simulink model "Model_XInput_wFeedback_Masked"  (R2023a)
settings: Solver=FixedStepAuto  StartTime=0.0  StopTime=100  FixedStep=0.01  RelTol=1e-3
settings Model: Creator=Mathias Voigt  LastModifiedBy=FIRSTMentor
settings SolverCC: AlgebraicLoopSolver=TrustRegion
settings DebuggingCC: UnconnectedInputMsg=warning  UnconnectedOutputMsg=warning  UnconnectedLineMsg=warning
settings ModelReferenceCC: EnableRefExpFcnMdlSchedulingChecks=on
settings SFSimCC: CustomCodeUndefinedFunction=UseInterfaceOnly

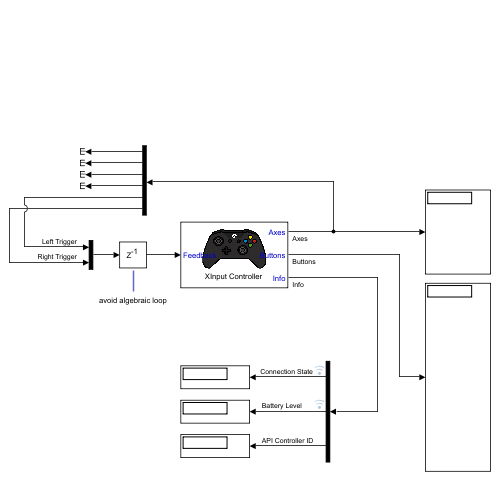
[thumbnail: Simulink's stored preview of the top-level diagram]
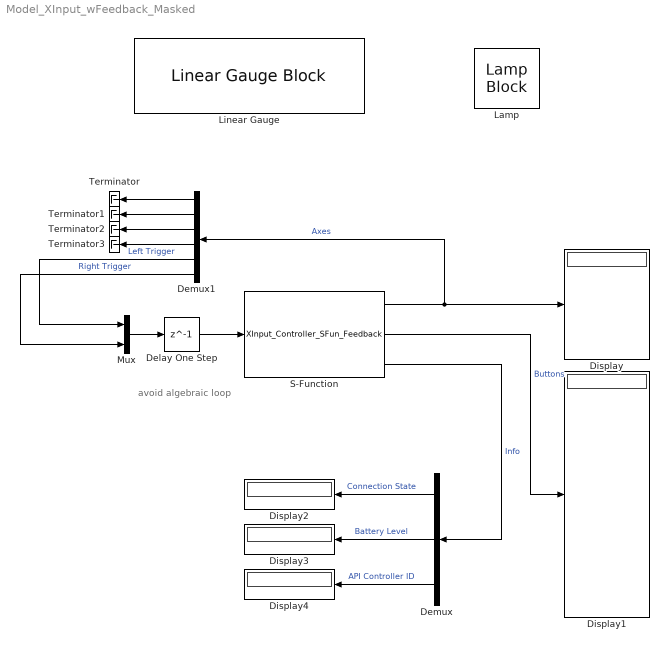
== system Model_XInput_wFeedback_Masked ==
  note: avoid algebraic loop
  Delay One Step : Delay  DelayLength=1
  Demux : Demux  Outputs=3
  Demux1 : Demux  Outputs=6
  Display{,1..4} (5 alike) : Display
  Lamp : LampBlock
  Linear Gauge : LinearGaugeBlock  TickInterval=25
  Mux : Mux  Inputs=2
  S-Function : S-Function  FunctionName=XInput_Controller_SFun_Feedback  Parameters=1  SFunctionDeploymentMode=off  EnableBusSupport=off  mask(XInput Controller (with Feedback)){ControllerID=1}
      mask help:
      | This Block will allow you to use XInput Controllers in Simulink.
      | XInput is the most Supported API.
      | Works with XBOX 360 and XBOX ONE Controllers.
      |
      | Use 'DEMUX' to access Signals
      | Output_1 [1x6]
      |   Analog Left X, Analog Left Y,
      |   Analog Right X, Analog Right Y,
      |   Left Trigger, Right Trigger
      | Output_2 [1x14]
      |   Up, Down, Left, Right,
      |   Start, Back, Left Stick, Right Stick,
      |   Left Shoulder, Right Shoulder,
      |   A, B, X, Y
      | Output_3 [1x3]
      |   Connection State, Battery Level (1-4), Controller ID
      | Input_1 [1x2]
      |   Left Motor, Right Motor (Force Feedback)
      mask init:
      | ControllerID;   
      | blk = gcb; 
      | get_String = get_param(blk,'ControllerID');
      | ControllerID = str2double(get_String);
      mask Help:
      | Based on Microsoft XInput API
      | Therefore the maximum of conneced Gamepads per PC is 4. First Gamepad has Controller ID 1.
      | 
      | Reference:
      | https://docs.microsoft.com/en-us/windows/win32/api/_xinput/
      | 
      | Tutorial:
      | https://docs.microsoft.com/en-us/windows/win32/xinput/getting-started-with-xinput
      | 
      | Info:
      | The Analog Sticks Deadzone is coded to:
      | Deadzone = 6144;
      | 0 <= Deadzone <= 65534
      | This is smaller then Microsoft default.
      | 
      | created by Mathias Voigt
      | Technische Universität Dresden
      | 2019
      mask TypeOptions ControllerID: 1 | 2 | 3 | 4
      mask DialogControl ParameterGroupVar Prompt: Controller ID
      mask Display:
      | %% Set Block picture from user Data
      | %  (permanent, picture file not needed)
      | %  see persistent_image_allocation.m
      | 
      | %get the picture data
      | UserDataStrut = get_param(gcb, 'UserData');
      | image(UserDataStrut.Image, [0.2, 0.3, 0.6, 0.6])
      | 
      | 
      | 
      | % conventional method (does not save picture data in Simulink)
      | % image('XBOX_One_Controller_Icon.png', [0.2, 0.3, 0.6, 0.6])
      | 
      | %% Create Port Labels
      | color('blue');
      | port_label('output', 1, 'Axes');
      | port_label('output', 2, 'Buttons');
      | port_label('output', 3, 'Info');
      | port_label('input',  1, 'Feedback');
      | 
      | %% Create S-Function Block Name
      | color('black');
      | text(0.5, 0.1, 'XInput Controller',...
      |      'horizontalAlignment', 'center',...
      |      'verticalAlignment', 'bottom');
  Terminator{,1..3} (4 alike) : Terminator
  wires:
  S-Function/2 -> Display1/1  "Buttons"
  S-Function/1 -> Demux1/1, Display/1  "Axes"
  Demux/1 -> Display2/1  "Connection State"
  Demux/2 -> Display3/1  "Battery Level"
  Demux/3 -> Display4/1  "API Controller ID"
  S-Function/3 -> Demux/1  "Info"
  Delay One Step/1 -> S-Function/1
  Mux/1 -> Delay One Step/1
  Demux1/6 -> Mux/2  "Right Trigger"
  Demux1/5 -> Mux/1  "Left Trigger"
  Demux1/1 -> Terminator/1
  Demux1/2 -> Terminator1/1
  Demux1/3 -> Terminator2/1
  Demux1/4 -> Terminator3/1
